simulink model "Lab7_p2_Motor_StepResp_13b"  (R2013b)
settings: Solver=FixedStepDiscrete  SolverMode=SingleTasking  StartTime=0.0  StopTime=inf  FixedStep=0.03  RelTol=1e-3
libraries: arduinolib x3, simulink x1
settings Model: SimulationMode=external  ExtModeTrigDuration=2  Creator=nding  LastModifiedBy=nding
settings OptimizationCC: OptimizeModelRefInitCode=on  LifeSpan=1
settings DebuggingCC: SolverPrmCheckMsg=none
settings HardwareCC: ProdBitPerInt=16  ProdBitPerPointer=8  ProdIntDivRoundTo=Zero  ProdEndianess=LittleEndian  ProdWordSize=8  ProdHWDeviceType=Atmel->AVR
settings RTWCC: SystemTargetFile=realtime.tlc  GenerateMakefile=off  TemplateMakefile=realtime.tmf  Description=Run on Target Hardware  RTWVerbose=off  ProcessScript=realtime_make_rtw_hook
settings STFCustomTargetCC: TargetLibSuffix=.a  GenerateSampleERTMain=on  ERTCustomFileBanners=on  SupportNonInlinedSFcns=off  SupportVariableSizeSignals=on  MATLABClassNameForMDSCustomization=Simulink.SoftwareTarget.ERTCustomization  GRTInterface=off  SystemTargetFile=realtime.tlc
settings ERTTargetCC: CodeReplacementLibrary=ANSI_C  GenerateSampleERTMain=on  ParMdlRefBuildCompliant=off  CompOptLevelCompliant=off  ConcurrentExecutionCompliant=off  CombineOutputUpdateFcns=off  ERTFirstTimeCompliant=off  SupportContinuousTime=on  SupportVariableSizeSignals=on  ModelStepFunctionPrototypeControlCompliant=off  CPPClassGenCompliant=off  ExtMode=on  ExtModeTransport=3  ExtModeMexArgs=0 11 115200 30  InlinedParameterPlacement=NonHierarchical  ERTSrcFileBannerTemplate=realtime_code_template.cgt  ERTHdrFileBannerTemplate=realtime_code_template.cgt  ERTDataSrcFileTemplate=realtime_code_template.cgt  ERTDataHdrFileTemplate=realtime_code_template.cgt  ERTCustomFileTemplate=realtime_file_process.tlc

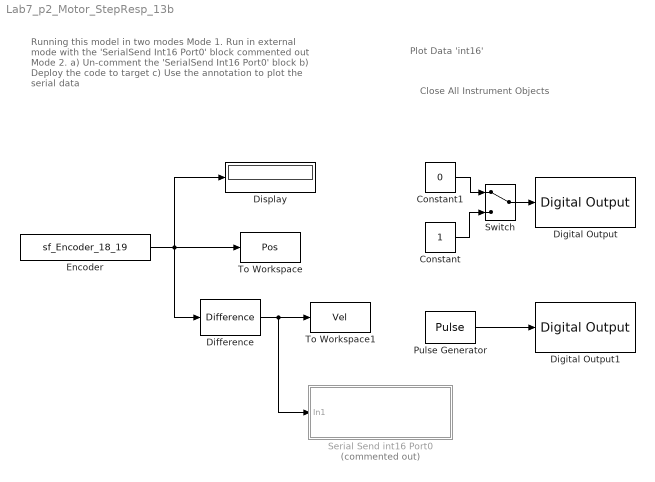
== system Lab7_p2_Motor_StepResp_13b ==
  note: Running this model in two modes
      | Mode 1. Run in external mode with the 'SerialSend Int16
      |               Port0' block commented out
      |
      | Mode 2. a) Un-comment the 'SerialSend Int16 Port0' block
      |               b) Deploy the code to target
      |               c) Use the annotation to plot the serial data
  note: Close All
      | Instrument Objects
  note: Plot Data 'int16'
  Constant : Constant
  Constant1 : Constant  Value=0
  Difference : simulink/Discrete/Difference  ICPrevInput=0.0  InputProcessing=Inherited  OutMin=[]  OutMax=[]  OutDataType=fixdt(1, 16)  OutScaling=2^-10  DoSatur=off
  Digital Output : arduinolib/Digital Output  pinNumber=44
  Digital Output1 : arduinolib/Digital Output  pinNumber=45
  Display : Display
  Encoder : S-Function  InitFcn=try, set_param(gcb,'FunctionName','sf_Encoder_18_19'), end  FunctionName=sf_Encoder_18_19  Parameters=uint8(0),uint8(18),uint8(19)  SFunctionModules=sf_Encoder_18_19_wrapper  EnableBusSupport=off  mask(S-Function Builder){}
      mask init:
      | val = [[.9  0.75 0.75 1 1 .9 .9 1]',[1 1 0.75 0.75 .9 .9 1 .9]'];try , sys = get_param(gcb,'SfunBuilderFcnName');if isempty(sys), sys = get_param(gcb,'FunctionName'); end,catch, sys = get_param(gcb,'FunctionName'); end
      settings: CopyFcn=set_param(gcbh,'LinkStatus','none')  PreSaveFcn=try, set_param(gcb,'FunctionName','sf_Encoder_18_19'), end  OpenFcn=sfunctionwizard(gcbh)
      mask Display: plot(val(:,1),val(:,2)),disp(sys), port_label('output',1,'pos')
  Pulse Generator : DiscretePulseGenerator  Period=120  PulseWidth=30  SampleTime=-1
  Serial Send int16 Port0 : Subsystem  Commented=on
  Switch : ManualSwitch
  To Workspace : ToWorkspace  VariableName=Pos  SampleTime=-1
  To Workspace1 : ToWorkspace  VariableName=Vel  SampleTime=-1
  wires:
  Encoder/1 -> To Workspace/1, Difference/1, Display/1
  Difference/1 -> Serial Send int16 Port0/1(In1), To Workspace1/1
  Switch/1 -> Digital Output/1
  Constant/1 -> Switch/2
  Constant1/1 -> Switch/1
  Pulse Generator/1 -> Digital Output1/1

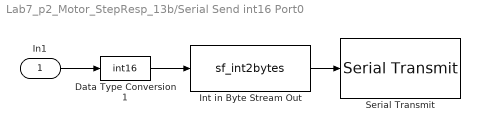
== system Lab7_p2_Motor_StepResp_13b/Serial Send int16 Port0 ==
  In1 : Inport
  Data Type Conversion1 : DataTypeConversion  OutDataTypeStr=int16
  Int in Byte Stream Out : S-Function  InitFcn=try, set_param(gcb,'FunctionName','sf_int2bytes'), end  FunctionName=sf_int2bytes  SFunctionModules=sf_int2bytes_wrapper  EnableBusSupport=off  mask(S-Function Builder){}
      mask init: same as Lab7_p2_Motor_StepResp_13b/Encoder
      settings: CopyFcn=set_param(gcb,'LinkStatus','none')  PreSaveFcn=try, set_param(gcb,'FunctionName','sf_int2bytes'), end  OpenFcn=sfunctionwizard(gcbh)
      mask Display: plot(val(:,1),val(:,2)),disp(sys), port_label('input',1,'int_in'), port_label('output',1,'bout')
  Serial Transmit : arduinolib/Serial Transmit  portNumber=0
  wires:
  Data Type Conversion1/1 -> Int in Byte Stream Out/1
  Int in Byte Stream Out/1 -> Serial Transmit/1
  In1/1 -> Data Type Conversion1/1
